simulink model "si_hydrostatic_si"  (R2025b)
settings: Solver=ode45  StartTime=0.0  StopTime=6  MaxStep=.002  RelTol=1e-9  AbsTol=1e-10
model workspace (MAT data in the model file):
  command_data = [0 0.002 0.004 0.006 0.008 0.01 0.012 0.014 0.016 0.018 0.02 0.022 ... (9003 elements, 3001x3)]
  p.pump_m3_per_rad = 2.30774667483e-05
  p.motor_m3_per_rad = 2.70563403256e-05
  p.capacitance_m3_per_pa = 1.8408e-12
  p.leakage_m3_per_s_pa = 1.4e-15
  p.vehicle_inertia_kg_m2 = 16512
  p.cardan_damping_nm_s = 0.33
  p.gear_ratio = -6.12
  p.axle_ratio = -23.3
  p.gearbox_efficiency = 0.98
  p.motor_efficiency = 0.697
  p.pump_time_constant_s = 0.13
  p.motor_time_constant_s = 0.22
  xinit = [0.25; 0.8; 2400209.42822; 47.9777859313]
settings Model: Creator=runner  LastModifiedBy=runner
settings DataIOCC: OutputOption=SpecifiedOutputTimes  OutputTimes=0:.01:6

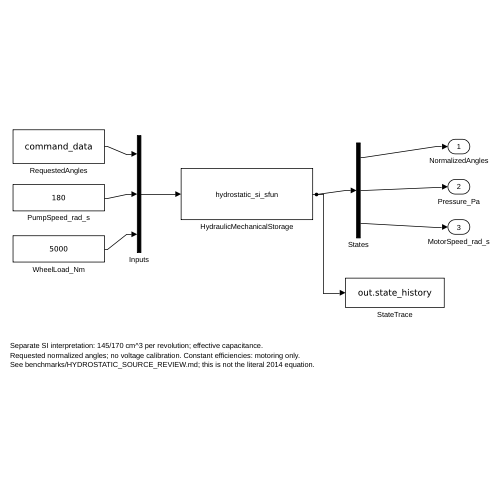
[thumbnail: Simulink's stored preview of the top-level diagram]
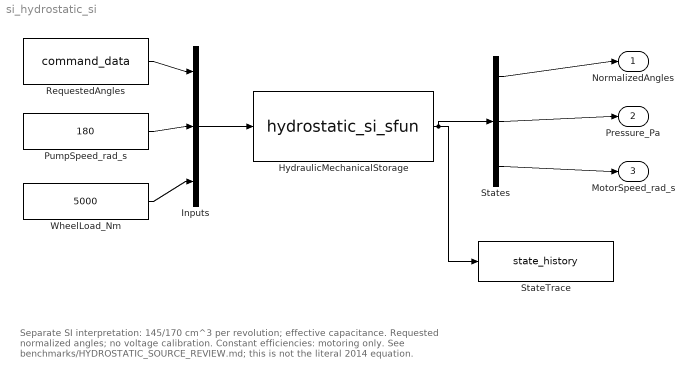
== system si_hydrostatic_si ==
  note: Separate SI interpretation: 145/170 cm^3 per revolution; effective capacitance.
      | Requested normalized angles; no voltage calibration. Constant efficiencies: motoring only.
      | See benchmarks/HYDROSTATIC_SOURCE_REVIEW.md; this is not the literal 2014 equation.
  HydraulicMechanicalStorage : M-S-Function  FunctionName=hydrostatic_si_sfun  Parameters=xinit,p
  Inputs : Mux  Inputs=3
  PumpSpeed_rad_s : Constant  Value=180
  RequestedAngles : FromWorkspace  VariableName=command_data
  StateTrace : ToWorkspace  VariableName=state_history  SaveFormat=Structure With Time  SampleTime=-1
  States : Demux  Outputs=[2 1 1]
  WheelLoad_Nm : Constant  Value=5000
  NormalizedAngles : Outport
  Pressure_Pa : Outport  Port=2
  MotorSpeed_rad_s : Outport  Port=3
  wires:
  States/1 -> NormalizedAngles/1
  States/2 -> Pressure_Pa/1
  States/3 -> MotorSpeed_rad_s/1
  RequestedAngles/1 -> Inputs/1
  PumpSpeed_rad_s/1 -> Inputs/2
  WheelLoad_Nm/1 -> Inputs/3
  Inputs/1 -> HydraulicMechanicalStorage/1
  HydraulicMechanicalStorage/1 -> States/1, StateTrace/1
